simulink model "Position_controller_demo_dex35_test"  (R2013a)
settings: Solver=ode4  SolverMode=SingleTasking  StartTime=0.0  StopTime=inf  FixedStep=0.0005  RelTol=1e-3
StartFcn:
  |  warndlg('Dexterit-E models cannot run under simulation. Please compile your model and run it from within Dexterit-E.');set_param(bdroot,'SimulationCommand','stop')
model workspace (MAT data in the model file):
  BKIN_STEP_TIME = 0.0005
  col_x = 1
  col_y = 2
  VRAD = 3
  COLOR = 4
  LOAD = 2
  MAX_MOVE_TIME = 4
  TARGET_COL = 1
  TRAJ_DURATION_COL = 3
libraries: General x3, KINARM_loads x2, KINARM_EP_loads x2, Video x2, KINARM_general x1, simulink x1
CloseFcn:
  | rtwprivate ssgencode ModelCloseRequest b2lab2d
settings Model: ModifiedComment=chris -- Wed Feb 16 09:18:30 2005 -- Version 1.1384  ModifiedHistory=Feb 16/05 - Add error repeat, add offset ramp  ExtModeArmWhenConnect=off  ExtModeLogAll=off  BufferReuse=off  Creator=Chris Grebeldinger  LastModifiedBy=BKIN TECHNOLOGIES
settings DataIOCC: LimitDataPoints=off  SignalLoggingSaveFormat=ModelDataLogs  SaveOutput=off  SaveTime=off  SignalLoggingName=sigsOut
settings OptimizationCC: BlockReduction=off  BooleanDataType=off  OptimizeBlockIOStorage=off  BufferReuse=off  ExpressionFolding=off  ExpressionDepthLimit=2147483647  FoldNonRolledExpr=off  LocalBlockOutputs=off  InitFltsAndDblsToZero=on
settings DebuggingCC: SaveWithParameterizedLinksMsg=none  SignalResolutionControl=TryResolveAllWithWarning  SolverPrmCheckMsg=none  MultiTaskDSMMsg=warning  MultiTaskCondExecSysMsg=none  FcnCallInpInsideContextMsg=UseLocalSettings  StrictBusMsg=None
settings HardwareCC: ProdIntDivRoundTo=Zero  ProdEndianess=LittleEndian  ProdHWDeviceType=Generic->32-bit x86 compatible  TargetHWDeviceType=32-bit Generic
settings SFSimCC: SimParseCustomCode=off
settings RTWCC: SystemTargetFile=xpctarget.tlc  TemplateMakefile=xpc_default_tmf  Description=xPC Target  ProcessScript=xpctarget_make_rtw_hook  IncludeERTFirstTime=on  RTWCompilerOptimization=On
settings CodeAppCC: MaxIdLength=63
settings xpcTargetCC: TargetFcnLib=ansi_tfl_tmw.mat  CodeReplacementLibrary=XPC_BLAS  ParMdlRefBuildCompliant=on  ConcurrentExecutionCompliant=on  CombineSignalStateStructs=off  MATLABClassNameForMDSCustomization=xpcAperiodicCustomization  GRTInterface=on  GenerateAllocFcn=off  xPCTaskExecutionProfile=off  xPCRL32EventNumber=5000  xPCisDownloadable=off  xPCLoadParamSetFile=off  xPCConcurrentTasks=off  xPCEnableSFAnimation=off

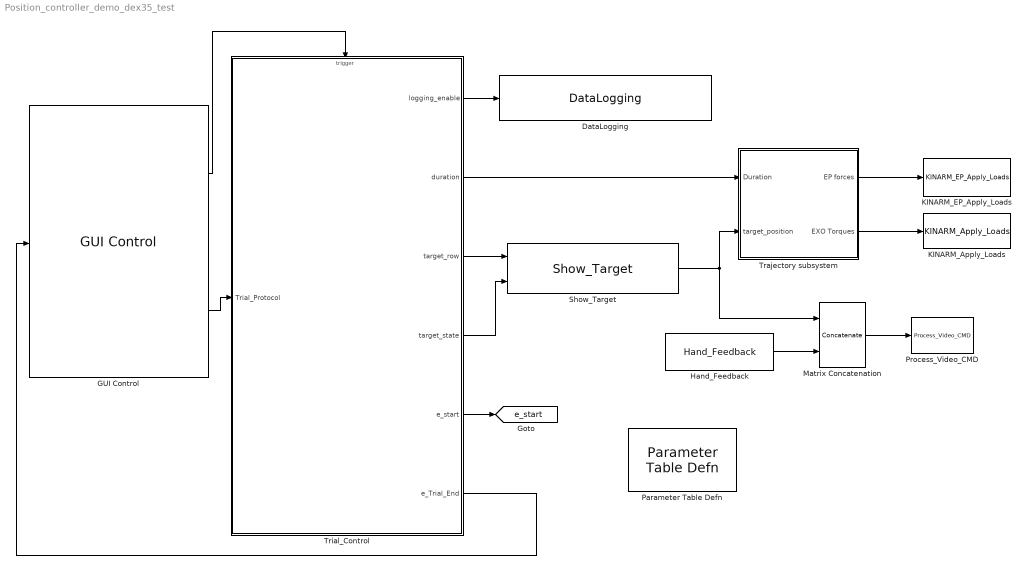
== system Position_controller_demo_dex35_test ==
  DataLogging : General/DataLogging  log_event_codes=off  log_analog_inputs=off
      link override Poll KINARM/EPTorqueCMD: GotoTag=KINARMEPTorqueCMD
      link override Poll KINARM/TorqueCMD: GotoTag=KINARMTorqueCMD
  GUI Control : General/GUI Control  target_type_str=Circle  Target_Type=1  XYcols=[1 2]  Vcols=3  Lcols=4  indices_padding=[0 0 0 0;0 0 0 0]  task_version=1.0  show_repeat_trial_flag=off
  Hand_Feedback : KINARM_general/Hand_Feedback  feedback_cntl_src=none
  KINARM_Apply_Loads : KINARM_loads/KINARM_Apply_Loads  up_duration=1500  down_duration=1500  max_torque=10
  KINARM_EP_Apply_Loads : KINARM_EP_loads/KINARM_EP_Apply_Loads  up_duration=1500  down_duration=1500  max_force=60
  Matrix Concatenation : Concatenate  Mode=Multidimensional array
  Parameter Table Defn : General/Parameter Table Defn  ShowInLibBrowser=0
  Process_Video_CMD : Video/Process_Video_CMD
  Show_Target : Video/Show_Target  target_type=Circle  num_states=1  attribcol1=[COLOR 0 0 VRAD]  attribcol2=[5 0 0 3]  attribcol3=[0 0 0 0]  attribcol4=[0 0 0 0]  attribcol5=[0 0 24 0]  stateindices_padding=[0 0 0 0 0 0 0;0 0 0 0 0 0 0;0 0 0 0 0 0 0;0 0 0 0 0 0 0;0 0 0 0 0 0 0]  source=dialog  opacity=100  target_display=Both subject and operator displays  num_col=4
  Trajectory subsystem : Subsystem
  Trial_Control : Stateflow chart  TreatAsAtomicUnit=on
  tag scope: e_start=global
  wires:
  Show_Target/1 -> Matrix Concatenation/1, Trajectory subsystem/2(target_position)
  Trial_Control/6(e_Trial_End) -> GUI Control/1
  GUI Control/1 -> Trial_Control/Trigger
  Trial_Control/4(target_state) -> Show_Target/2
  Trial_Control/3(target_row) -> Show_Target/1
  Matrix Concatenation/1 -> Process_Video_CMD/1
  Hand_Feedback/1 -> Matrix Concatenation/2
  GUI Control/2 -> Trial_Control/1(Trial_Protocol)
  Trial_Control/1(logging_enable) -> DataLogging/1
  Trial_Control/2(duration) -> Trajectory subsystem/1(Duration)
  Trajectory subsystem/1(EP forces) -> KINARM_EP_Apply_Loads/1
  Trajectory subsystem/2(EXO Torques) -> KINARM_Apply_Loads/1
  Trial_Control/5(e_start) -> [e_start]

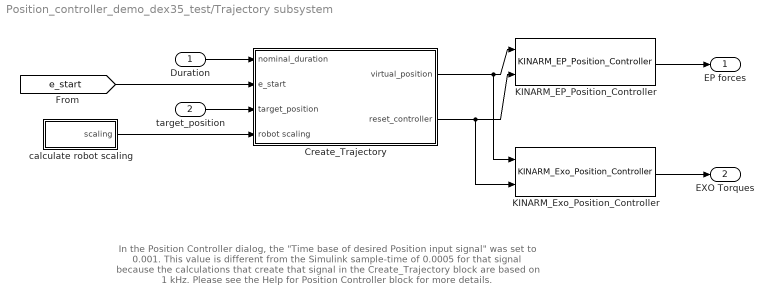
== system Position_controller_demo_dex35_test/Trajectory subsystem ==
  note: In the Position Controller dialog, the "Time base of desired Position input signal" was set to 0.001.
      | This value is different from the Simulink sample-time of 0.0005 for that signal because the calculations
      | that create that signal in the Create_Trajectory block are based on 1 kHz. Please see the Help for
      | Position Controller block for more details.
  Duration : Inport
  target_position : Inport  Port=2
  Create_Trajectory : Subsystem
  KINARM_EP_Position_Controller : KINARM_EP_loads/KINARM_EP_Position_Controller  use_dom_hand=on  inertias_for_FF=KINARM End Point robot  gain_choice=Standard Movement  sample_time=0.001
  KINARM_Exo_Position_Controller : KINARM_loads/KINARM_Exo_Position_Controller  use_dom_hand=on  KINARM_Type=Human  inertias_for_FF=KINARM robot  angles_or_XY=End-point (global x/y)  sample_time=0.001
  calculate robot scaling : Subsystem
  EP forces : Outport
  EXO Torques : Outport  Port=2
  wires:
  Create_Trajectory/2(reset_controller) -> KINARM_EP_Position_Controller/2, KINARM_Exo_Position_Controller/2
  Create_Trajectory/1(virtual_position) -> KINARM_EP_Position_Controller/1, KINARM_Exo_Position_Controller/1
  KINARM_EP_Position_Controller/1 -> EP forces/1
  KINARM_Exo_Position_Controller/1 -> EXO Torques/1
  target_position/1 -> Create_Trajectory/3(target_position)
  Duration/1 -> Create_Trajectory/1(nominal_duration)
  [e_start] -> Create_Trajectory/2(e_start)
  calculate robot scaling/1(scaling) -> Create_Trajectory/4(robot scaling)

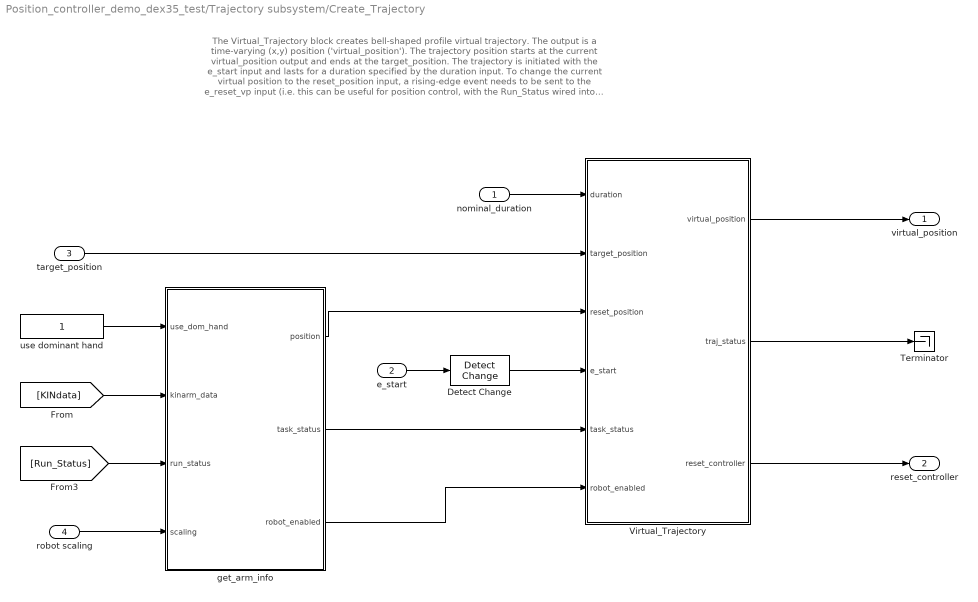
== system Position_controller_demo_dex35_test/Trajectory subsystem/Create_Trajectory ==
  note: The Virtual_Trajectory block creates bell-shaped profile virtual trajectory.
      | The output is a time-varying (x,y) position ('virtual_position').
      |
      | The trajectory position starts at the current virtual_position output and ends at the target_position.
      | The trajectory is initiated with the e_start input and lasts for a duration specified by the duration input.
      |
      | To change the current virtual position to the reset_position input, a rising-edge event needs to be sent to the e_reset_vp input
      | (i.e. this can be useful for position control, with the Run_Status wired into the e_reset input).
      | If such an event occurs during a virtual trajectory, the trajectory is halted immediately.
  nominal_duration : Inport
  e_start : Inport  Port=2
  target_position : Inport  Port=3
  robot scaling : Inport  Port=4
  Detect Change : simulink/Logic and Bit Operations/Detect Change  vinit=0  InputProcessing=Inherited  OutDataTypeStr=uint8
  Terminator : Terminator
  Virtual_Trajectory : Subsystem
  get_arm_info : MATLAB Function  TreatAsAtomicUnit=on
  use dominant hand : Constant
  virtual_position : Outport
  reset_controller : Outport  Port=2
  wires:
  Virtual_Trajectory/1(virtual_position) -> virtual_position/1
  nominal_duration/1 -> Virtual_Trajectory/1(duration)
  e_start/1 -> Detect Change/1
  target_position/1 -> Virtual_Trajectory/2(target_position)
  Detect Change/1 -> Virtual_Trajectory/4(e_start)
  use dominant hand/1 -> get_arm_info/1(use_dom_hand)
  [KINdata] -> get_arm_info/2(kinarm_data)
  get_arm_info/1(position) -> Virtual_Trajectory/3(reset_position)
  Virtual_Trajectory/3(reset_controller) -> reset_controller/1
  get_arm_info/2(task_status) -> Virtual_Trajectory/5(task_status)
  get_arm_info/3(robot_enabled) -> Virtual_Trajectory/6(robot_enabled)
  [Run_Status] -> get_arm_info/3(run_status)
  Virtual_Trajectory/2(traj_status) -> Terminator/1
  robot scaling/1 -> get_arm_info/4(scaling)

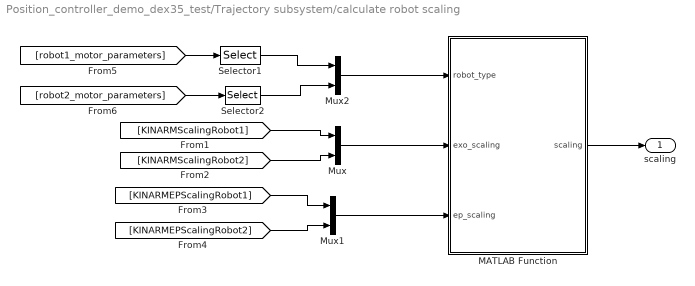
== system Position_controller_demo_dex35_test/Trajectory subsystem/calculate robot scaling ==
  MATLAB Function : MATLAB Function  TreatAsAtomicUnit=on
  Mux : Mux  Inputs=2
  Mux1 : Mux  Inputs=2
  Mux2 : Mux  Inputs=2
  Selector1 : Selector  InputPortWidth=9  IndexOptions=Index vector (dialog)  Indices=[7]  OutputSizes=[(-2)]
  Selector2 : Selector  InputPortWidth=9  IndexOptions=Index vector (dialog)  Indices=[7]  OutputSizes=[(-2)]
  scaling : Outport
  wires:
  [KINARMScalingRobot1] -> Mux/1
  [KINARMScalingRobot2] -> Mux/2
  Mux/1 -> MATLAB Function/2(exo_scaling)
  Mux1/1 -> MATLAB Function/3(ep_scaling)
  Mux2/1 -> MATLAB Function/1(robot_type)
  MATLAB Function/1(scaling) -> scaling/1
  [robot2_motor_parameters] -> Selector2/1
  Selector2/1 -> Mux2/2
  [KINARMEPScalingRobot2] -> Mux1/2
  [KINARMEPScalingRobot1] -> Mux1/1
  Selector1/1 -> Mux2/1
  [robot1_motor_parameters] -> Selector1/1

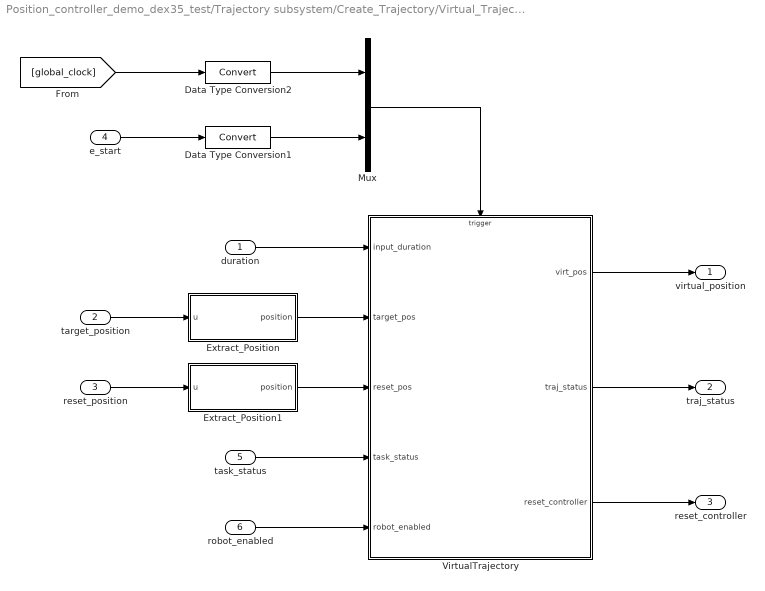
== system Position_controller_demo_dex35_test/Trajectory subsystem/Create_Trajectory/Virtual_Trajectory ==
  duration : Inport
  target_position : Inport  Port=2
  reset_position : Inport  Port=3
  e_start : Inport  Port=4
  task_status : Inport  Port=5
  robot_enabled : Inport  Port=6
  Data Type Conversion1 : DataTypeConversion
  Data Type Conversion2 : DataTypeConversion
  Extract_Position : MATLAB Function  TreatAsAtomicUnit=on
  Extract_Position1 : MATLAB Function  TreatAsAtomicUnit=on
  Mux : Mux  Inputs=2
  VirtualTrajectory : Stateflow chart  TreatAsAtomicUnit=on
  virtual_position : Outport
  traj_status : Outport  Port=2
  reset_controller : Outport  Port=3
  wires:
  e_start/1 -> Data Type Conversion1/1
  target_position/1 -> Extract_Position/1(u)
  [global_clock] -> Data Type Conversion2/1
  Mux/1 -> VirtualTrajectory/Trigger
  duration/1 -> VirtualTrajectory/1(input_duration)
  VirtualTrajectory/1(virt_pos) -> virtual_position/1
  Extract_Position/1(position) -> VirtualTrajectory/2(target_pos)
  reset_position/1 -> Extract_Position1/1(u)
  Data Type Conversion2/1 -> Mux/1
  VirtualTrajectory/2(traj_status) -> traj_status/1
  robot_enabled/1 -> VirtualTrajectory/5(robot_enabled)
  task_status/1 -> VirtualTrajectory/4(task_status)
  Data Type Conversion1/1 -> Mux/2
  Extract_Position1/1(position) -> VirtualTrajectory/3(reset_pos)
  VirtualTrajectory/3(reset_controller) -> reset_controller/1

== stateflow chart Position_controller_demo_dex35_test/Trial_Control ==
  settings: sampleTime=0.001
  state Main_Trial
    state StayCentre/
      target_row = Trial_Protocol[TARGET_COL];
      target_state = 1;
      logging_enable = 1;
      duration =Trial_Protocol[TRAJ_DURATION_COL];
      max_move_time = Trial_Protocol[MAX_MOVE_TIME];
    state MoveLoadedArm/
      e_start;
    state EndOfTrial/
      target_state = 0;
      logging_enable = 0;
    StayCentre -> MoveLoadedArm : after(2, e_clk)
    MoveLoadedArm -> EndOfTrial : after(duration, e_clk)
  state init/
  state Inter_Trial_State/
    e_Trial_End
  state WaitForFlagToSet
  (default) -> init
  init -> StayCentre
  Inter_Trial_State -> StayCentre
  WaitForFlagToSet -> Inter_Trial_State : after(2, e_clk)
  Main_Trial -> WaitForFlagToSet [order 2] : e_ExitTrialNow/
      | target_state = 0;
      | logging_enable = 0;
      | tickCount = 10;
  Main_Trial -> Inter_Trial_State [order 1] : after(max_move_time, e_clk)
  data: logging_enable output boolean; duration output double; target_row output [1..32]; target_state output double; tickCount local double; Trial_Protocol input double; max_move_time local double size=1
  data target_row settings: description=index of the row currently being used in the TargetTable
  events: e_start output EITHER_EDGE_EVENT; e_clk input RISING_EDGE_EVENT; e_ExitTrialNow input EITHER_EDGE_EVENT; e_Trial_End output EITHER_EDGE_EVENT

== matlab function Position_controller_demo_dex35_test/Trajectory subsystem/calculate robot scaling/MATLAB Function ==
  data: robot_type input; scaling output; exo_scaling input; ep_scaling input
function scaling = fcn(robot_type, exo_scaling, ep_scaling)
%#codegen

scaling = [0, 0];

%0 = EXO, 1 = EP, 2 = NHP
for n=1:2
    if robot_type(n) == 1
        scaling(n) = ep_scaling(n);
    else
        scaling(n) = exo_scaling(n);
    end
end

== matlab function Position_controller_demo_dex35_test/Trajectory subsystem/Create_Trajectory/Virtual_Trajectory/Extract_Position ==
  settings: fimath=|
      | fimath(...
      | 'RoundMode', 'floor',...
      | 'OverflowMode', 'wrap',...
      | 'ProductMode', 'KeepLSB', 'ProductWordLength', 32,...
      | 'SumMode', 'KeepLSB', 'SumWordLength', 32,...
      | 'CastBeforeSum', false)
  data: u input; position output
function position = fcn(u)

position=[0,0];	%initialization
if length(u)==2	%input is assumed to be (x,y) position, global coordinates, (m)		
	position=u;
else			%input is assumed to be a VCODE
	position(1)=u(3);
	position(2)=u(4);
end

== matlab function Position_controller_demo_dex35_test/Trajectory subsystem/Create_Trajectory/Virtual_Trajectory/Extract_Position1 ==
  settings: fimath=|
      | fimath(...
      | 'RoundMode', 'floor',...
      | 'OverflowMode', 'wrap',...
      | 'ProductMode', 'KeepLSB', 'ProductWordLength', 32,...
      | 'SumMode', 'KeepLSB', 'SumWordLength', 32,...
      | 'CastBeforeSum', false)
  data: u input; position output
function position = fcn(u)

position=[0,0];	%initialization
if length(u)==2	%input is assumed to be (x,y) position, global coordinates, (m)		
	position=u;
else			%input is assumed to be a VCODE
	position(1)=u(3);
	position(2)=u(4);
end

== stateflow chart Position_controller_demo_dex35_test/Trajectory subsystem/Create_Trajectory/Virtual_Trajectory/VirtualTrajectory ==
  state Initialization/
    virt_pos = reset_pos;
    // this initialization ensures that the virtual position
    // starts off as something reasonable
    traj_status = 0;   // initialize trajectory status
  state main/
    state wait_for_trigger/
      reset_controller = 0;
    state wait_1_ms_b/
      // wait for controller
      // to be reset
    state on_ramp/
      entry: tick = 0;    // initialize the tick counter
      reset_controller = 0;
      final_pos = target_pos;   // set the final position of the trajectory
      start_pos = virt_pos;   // set the start position of the trajectory
      duration = input_duration;   // store the duration of the trajectory
      traj_status = 1;   // indicate an ongoing trajectory
      during:
      on e_clk: tick++;
      // the trajectory velocity will have a bell shaped profile
      trajectory_shape = tick/duration-sin(2*pi*tick/duration)/(2*pi);
      virt_pos[1] = start_pos[1] + (final_pos[1] - start_pos[1]) * trajectory_shape;
      virt_pos[2] = start_pos[2] + (final_pos[2] - start_pos[2]) * trajectory_shape;
    main -> wait_1_ms_b [order 1] : [(robot_enabled == 1) && (traj_status == -1)]/
        | traj_status = 1;
        | virt_pos = reset_pos;
        | reset_controller = 1;
        | // trajectory was halted and
        | //is now being re-started
    wait_for_trigger -> (junction 20) : e_start
    (junction 20) -> wait_for_trigger [order 2]
    wait_1_ms_b -> (junction 20) : after(1, e_clk)
    (junction 20) -> on_ramp [order 1] : [input_duration>0]
    on_ramp -> wait_for_trigger [order 2] : [robot_enabled == 0]/
        | traj_status = -1;
        | // robot disabled
    on_ramp -> wait_for_trigger [order 1] : after(duration, e_clk)/
        | traj_status = 0
        | // trajectory completed
  state wait_1_ms/
    // wait for controller
    // to be reset
  state task_not_running/
    // wait for task_status to change
    // keep updating virt_pos so that the feedback
    // controller output, which is filtered, does not become
    // huge, resulting in a 'bump' if we don't do this.
    traj_status = 0;
    reset_controller = 0;
    during:
    virt_pos = reset_pos;
  (default) -> Initialization
  Initialization -> wait_for_trigger
  wait_1_ms -> wait_for_trigger : after(1, e_clk)
  task_not_running -> wait_1_ms : [task_status > 0]/
      | reset_controller = 1;
      | // task is running again,
      | // so reset position controller
  main -> task_not_running [order 1] : [task_status == 0]/
      | // means that run_status == 0
      | // AND that torque scaling at
      | // end of task is finished
  data: input_duration input double; target_pos input double size=[1 2]; tick local double; duration local double; reset_pos input double size=[1 2]; task_status input double; pi constant double =3.14159265358979; trajectory_shape local double; virt_pos output double size=[1 2]; traj_status output double; robot_enabled input double; start_pos local double size=[1 2]; final_pos local double size=[1 2]; reset_controller output double
  events: e_clk input RISING_EDGE_EVENT; e_start input RISING_EDGE_EVENT

== matlab function Position_controller_demo_dex35_test/Trajectory subsystem/Create_Trajectory/get_arm_info ==
  settings: fimath=|
      | fimath(...
      | 'RoundMode', 'floor',...
      | 'OverflowMode', 'wrap',...
      | 'ProductMode', 'KeepLSB', 'ProductWordLength', 32,...
      | 'SumMode', 'KeepLSB', 'SumWordLength', 32,...
      | 'CastBeforeSum', false)
  data: position output; task_status output; use_dom_hand input; kinarm_data input; run_status input; scaling input; robot_enabled output
function [position, task_status, robot_enabled]  = fcn(use_dom_hand, kinarm_data, run_status, scaling)
%
% get current hand position and robot enabled status
%
% May 2009
%

hpx_index = 23;
hpy_index = 24;
robot_disabled_index = 37;

%determine which arm to apply the load to
dominant_hand=kinarm_data(3,1);						%kinarm_data(3,1) tells which arm is the dominant arm
if use_dom_hand == 1
	feedback_arm = dominant_hand;
else
	feedback_arm = 3 - dominant_hand;
end

hpx = kinarm_data( feedback_arm, hpx_index );
hpy = kinarm_data( feedback_arm, hpy_index );
position = [hpx hpy];

if kinarm_data( feedback_arm, robot_disabled_index ) == 0;
    robot_enabled = 1;
else
    robot_enabled = 0;
end

% if the task has stopped/paused (i.e. run_status == 0) AND the torques outputs
% have scaled down to 0, then set the task_status = 0.
if run_status == 0 && scaling(feedback_arm) == 0
    task_status = 0;
else
    task_status = 1;
end
